simulink model "FCEV_Hybrid_Powertrain_EMS"  (R2025b)
settings: Solver=FixedStepDiscrete  StartTime=0.0  StopTime=600  FixedStep=Ts  RelTol=1e-3
values from neighbouring files (symbols this model uses):
  P_fc_initial = 60    [FCEV_setup.m]
  SOC_initial = 0.60    (= 0.6)    [FCEV_setup.m]
  Ts = 0.1    [FCEV_drivecycle.m]    (also in FCEV_setup.m)
settings Model: Creator=raysu  LastModifiedBy=raysu

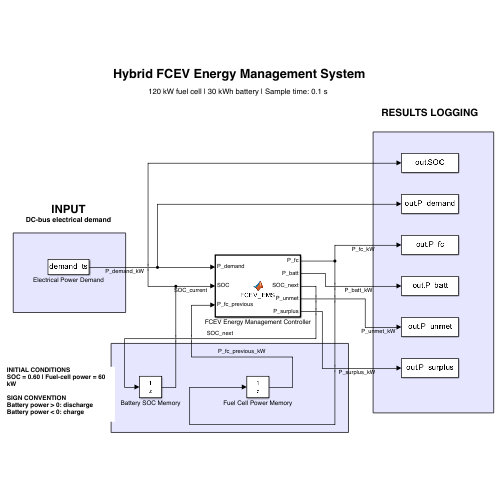
[thumbnail: Simulink's stored preview of the top-level diagram]
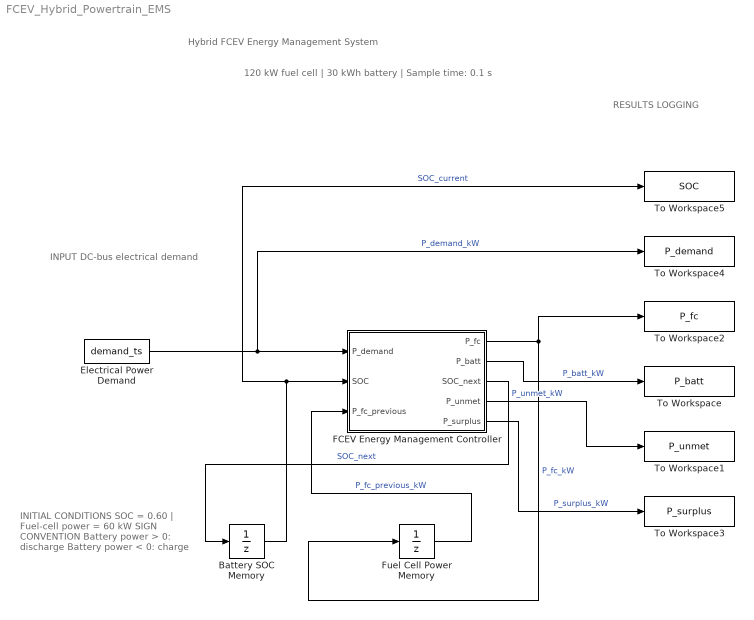
== system FCEV_Hybrid_Powertrain_EMS ==
  note: INITIAL CONDITIONS
      | SOC = 0.60 | Fuel-cell power = 60 kW
      |
      | SIGN CONVENTION
      | Battery power > 0: discharge
      | Battery power < 0: charge
  note: RESULTS LOGGING
  note: INPUT
      | DC-bus electrical demand
  note: 120 kW fuel cell | 30 kWh battery | Sample time: 0.1 s
  note: Hybrid FCEV Energy Management System
  Battery SOC Memory : UnitDelay  InitialCondition=SOC_initial  SampleTime=Ts  HasFrameUpgradeWarning=on
  Electrical Power Demand : FromWorkspace  VariableName=demand_ts  SampleTime=Ts  Interpolate=off  OutputAfterFinalValue=Holding final value
  FCEV Energy Management Controller : MATLAB Function  TreatAsAtomicUnit=on
  Fuel Cell Power Memory : UnitDelay  InitialCondition=P_fc_initial  SampleTime=Ts  HasFrameUpgradeWarning=on
  To Workspace : ToWorkspace  VariableName=P_batt  SaveFormat=Timeseries  SampleTime=-1
  To Workspace1 : ToWorkspace  VariableName=P_unmet  SaveFormat=Timeseries  SampleTime=-1
  To Workspace2 : ToWorkspace  VariableName=P_fc  SaveFormat=Timeseries  SampleTime=-1
  To Workspace3 : ToWorkspace  VariableName=P_surplus  SaveFormat=Timeseries  SampleTime=-1
  To Workspace4 : ToWorkspace  VariableName=P_demand  SaveFormat=Timeseries  SampleTime=-1
  To Workspace5 : ToWorkspace  VariableName=SOC  SaveFormat=Timeseries  SampleTime=-1
  wires:
  Electrical Power Demand/1 -> To Workspace4/1, FCEV Energy Management Controller/1(P_demand)  "P_demand_kW"
  Battery SOC Memory/1 -> To Workspace5/1, FCEV Energy Management Controller/2(SOC)  "SOC_current"
  Fuel Cell Power Memory/1 -> FCEV Energy Management Controller/3(P_fc_previous)  "P_fc_previous_kW"
  FCEV Energy Management Controller/1(P_fc) -> To Workspace2/1, Fuel Cell Power Memory/1  "P_fc_kW"
  FCEV Energy Management Controller/3(SOC_next) -> Battery SOC Memory/1  "SOC_next"
  FCEV Energy Management Controller/2(P_batt) -> To Workspace/1  "P_batt_kW"
  FCEV Energy Management Controller/4(P_unmet) -> To Workspace1/1  "P_unmet_kW"
  FCEV Energy Management Controller/5(P_surplus) -> To Workspace3/1  "P_surplus_kW"

== matlab function FCEV_Hybrid_Powertrain_EMS/FCEV Energy Management Controller ==
  data: P_demand input; P_fc output; SOC input; P_fc_previous input; P_batt output; SOC_next output; P_unmet output; P_surplus output
function [P_fc, P_batt, SOC_next, P_unmet, P_surplus] = ...
    FCEV_EMS(P_demand, SOC, P_fc_previous)
%#codegen
% All power values are DC-bus power in kW.
% Positive battery power = discharge.
% Negative battery power = charge.

%% Parameters
Ts = 0.1;
dt_h = Ts / 3600;

E_batt = 30;
eta_batt = 0.95;

SOC_min = 0.40;
SOC_max = 0.80;
SOC_ref = 0.60;

P_fc_max = 120;
P_fc_min = 10;
P_fc_ramp = 10;       % kW/s

P_batt_dis_max = 100;
P_batt_ch_max = 60;

tau_fc = 20;         % Fuel-cell smoothing time constant, s
K_soc = 200;         % SOC correction gain, kW per unit SOC

%% 1. Battery power available during this sample
P_dis_available = max(0, ...
    (SOC - SOC_min) * E_batt * eta_batt / dt_h);

P_ch_available = max(0, ...
    (SOC_max - SOC) * E_batt / (eta_batt * dt_h));

P_dis_limit = min(P_batt_dis_max, P_dis_available);
P_ch_limit = min(P_batt_ch_max, P_ch_available);

%% 2. Fuel-cell operating target
% SOC below reference increases requested fuel-cell power.
P_fc_target = max(P_demand, 0) + K_soc * (SOC_ref - SOC);

% Permit a simplified zero-power state.
if P_fc_target > 0
    P_fc_target = max(P_fc_target, P_fc_min);
end

P_fc_target = min(max(P_fc_target, 0), P_fc_max);

% Avoid requesting more FC power than load + charge acceptance.
% Ramp-down limits may still cause temporary surplus.
P_fc_target = min(P_fc_target, ...
    max(0, P_demand + P_ch_limit));

%% 3. Smooth response and apply ramp limit
alpha = Ts / (tau_fc + Ts);

P_fc_filtered = P_fc_previous + ...
    alpha * (P_fc_target - P_fc_previous);

max_change = P_fc_ramp * Ts;

P_fc = min(P_fc_filtered, P_fc_previous + max_change);
P_fc = max(P_fc, P_fc_previous - max_change);
P_fc = min(max(P_fc, 0), P_fc_max);

%% 4. Battery supplies or absorbs the residual
P_batt_requested = P_demand - P_fc;

P_batt = min(max(P_batt_requested, -P_ch_limit), ...
    P_dis_limit);

%% 5. Update stored battery energy
if P_batt >= 0
    SOC_next = SOC - ...
        P_batt * dt_h / (eta_batt * E_batt);
else
    SOC_next = SOC - ...
        P_batt * dt_h * eta_batt / E_batt;
end

% Numerical guard; available-power limits enforce the boundaries.
SOC_next = min(max(SOC_next, SOC_min), SOC_max);

%% 6. Account for residual power
P_balance = P_demand - P_fc - P_batt;

P_unmet = max(P_balance, 0);
P_surplus = max(-P_balance, 0);

end
